simulink model "ControlThreePhaseSolarInverter"  (R2025a)
settings: Solver=VariableStepAuto  StartTime=0.0  StopTime=T  RelTol=1e-3
PreLoadFcn:
  | run('ControlThreePhaseSolarInverterParameters.m');
values from neighbouring files (symbols this model uses):
  c = 10.5e-4    (= 0.00105)    [ControlThreePhaseSolarInverterParameters.m]
  l = 1e-3    (= 0.001)    [ControlThreePhaseSolarInverterParameters.m]
  Ts = 50e-6    (= 5e-05)    [ControlThreePhaseSolarInverterParameters.m]
undefined symbols (not defined in the file or in its folder): array, grid, mPPT, panel
libraries: nesl_utility x9, ee_lib x6, fl_lib x5, eeRenewablesControl x1
settings Model: Creator=The MathWorks, Inc.  LastModifiedBy=The MathWorks, Inc.
settings DataIOCC: ExternalInput=getinputstruct(op)  InitialState=getstatestruct(op)  ReturnWorkspaceOutputs=off  SignalLoggingName=logsout_PVControllerdemo
settings OptimizationCC: ReuseModelBlockBuffer=off
settings ModelReferenceCC: EnableRefExpFcnMdlSchedulingChecks=on
settings RTWCC: GPUComputeCapability=3.5
settings SimscapeCC: SimscapeLogType=all  SimscapeLogSimulationStatistics=on  SimscapeLogName=simlog_PVControllerdemo

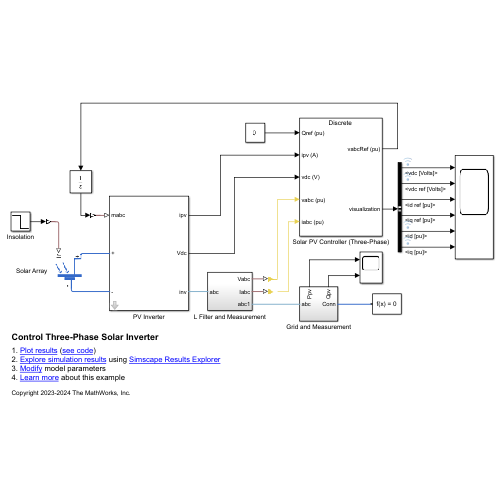
[thumbnail: Simulink's stored preview of the top-level diagram]
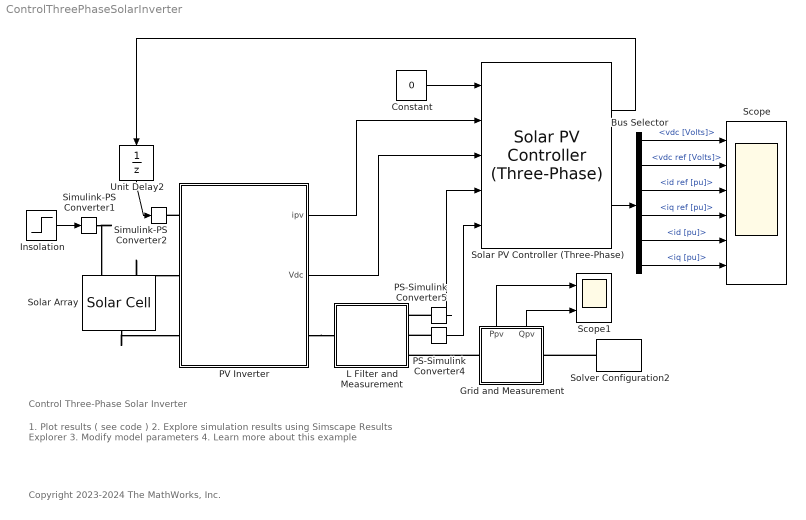
== system ControlThreePhaseSolarInverter ==
  note: 1. Plot results ( see code )
      | 2. Explore simulation results using Simscape Results Explorer
      | 3. Modify model parameters
      | 4. Learn more about this example
  note: Control Three-Phase Solar Inverter
  note: Copyright 2023-2024 The MathWorks, Inc.
  Bus Selector : BusSelector  OutputSignals=vdc [Volts],vdc ref [Volts],id ref [pu],iq ref [pu],id [pu],iq [pu]
  Constant : Constant  Value=0
  Grid and Measurement : Subsystem
      settings: PortSchema="{\"entries\":[{\"content\":{\"sides\":[{\"content\":{\"connectorIds\":[\"LConn1\"]},\"type\":\"ConnectorPlacement.EquallySpacedRectSide\",\"uuid\":\"53f3f0d9-a8a4-44c6-9152-358ba6ebb479\"},{\"content\":{\"connectorIds\":[\"RConn1\"],\"side\":\"RIGHT\"},\"type\":\"ConnectorPlacement.EquallySpacedRectSide\",\"uuid\":\"8260b293-3060-4415-851b-a3b9997b28bb\"},{\"content\":{\"connectorIds\":[\"Out1\",\"Out2\"],\"side\":\"TOP\"},\"type\":\"ConnectorPlacement.EquallySpacedRectSide\",\"uuid\":\"46e5815a-3c68-44c4-8def-43d274ad88a1\"}]},\"type\":\"ConnectorPlacement.EquallySpacedConnector\",\"uuid\":\"d7b5f747-a402-4a49-af60-c72c4c55231a\"}],\"packageUris\":[\"http://schema.mathworks.com/mf0/Connector/R2020b\"],\"version\":\"1.0\"}"
  Insolation : Step  Time=2  Before=1000  After=800  SampleTime=Ts
  L Filter and Measurement : Subsystem
  PS-Simulink Converter4 : nesl_utility/PS-Simulink Converter  PhysicalDomain=network_engine_domain  SubClassName=ps_output  LeftPortType=input  RightPortType=output  PseudoPeriodic=off  Frequencies=[]  VectorFormat=inherit  Unit=inherit  AffineConversion=off
  PS-Simulink Converter5 : nesl_utility/PS-Simulink Converter  PhysicalDomain=network_engine_domain  SubClassName=ps_output  LeftPortType=input  RightPortType=output  PseudoPeriodic=off  Frequencies=[]  VectorFormat=inherit  Unit=inherit  AffineConversion=off
  PV Inverter : Subsystem  mask{c=c, c_unit=F, g=0, g_unit=1/Ohm, vc_priority=None, vc_specify=on, vc=mPPT.initialVoltage, vc_unit=V, Pfixed=1, Pfixed_unit=W}
      mask prompts: c "Capacitance"; g "Parallel conductance"; vc_priority "Initial voltage priority"; vc_specify "Initial voltage"; vc "Initial vc"; Pfixed "Fixed power loss"
      mask TypeOptions c: Capacitor/c
      mask TypeOptions c_unit: Capacitor/c_unit
      mask TypeOptions g: Capacitor/g
      mask TypeOptions g_unit: Capacitor/g_unit
      mask TypeOptions vc_priority: Capacitor/vc_priority
      mask TypeOptions vc_specify: Capacitor/vc_specify
      mask TypeOptions vc: Capacitor/vc
      mask TypeOptions vc_unit: Capacitor/vc_unit
      mask TypeOptions Pfixed:
      | Average-Value
      | Voltage Source
      | Converter
      | (Three-Phase)/Pfixed
      mask TypeOptions Pfixed_unit:
      | Average-Value
      | Voltage Source
      | Converter
      | (Three-Phase)/Pfixed_unit
      mask DialogControl Container4 Prompt: DC Link Capacitance
      mask DialogControl Container5 Prompt: Average Inverter
  Scope : Scope  NumInputPorts=6
      settings: ActiveDisplayYMinimum=759.67451  ActiveDisplayYMaximum=881.42949
  Scope1 : Scope  NumInputPorts=2
      settings: ActiveDisplayYMinimum=-10224.92366  ActiveDisplayYMaximum=92024.31296
  Simulink-PS Converter1 : nesl_utility/Simulink-PS Converter  PhysicalDomain=network_engine_domain  SubClassName=ps_input  LeftPortType=input  RightPortType=output  PseudoPeriodic=off  Frequencies=[]  NoiseDistribution=none  NoiseParameters=[]  Unit=1  AffineConversion=off  FilteringAndDerivatives=provide  SimscapeFilterOrder=1  InputFilterTimeConstant=0.001  UdotUserProvided=0
  Simulink-PS Converter2 : nesl_utility/Simulink-PS Converter  PhysicalDomain=network_engine_domain  SubClassName=ps_input  LeftPortType=input  RightPortType=output  PseudoPeriodic=off  Frequencies=[]  NoiseDistribution=none  NoiseParameters=[]  Unit=1  AffineConversion=off  FilteringAndDerivatives=provide  SimscapeFilterOrder=1  InputFilterTimeConstant=0.001  UdotUserProvided=0
  Solar Array : ee_lib/Sources/Solar Cell  prm=3  Isc=3.8 A  Voc=0.586 V  Is=solarcell.diodeSaturationCurrent A  Is2=0 A  Iph=solarcell.solarGeneratedCurrent_AM A  Ir0=1000 W/m^2  ec=solarcell.qualityFactori  N2=solarcell.qualityFactorj  Rs=solarcell.seriesResistance Ohm  Rp=solarcell.parallelResistance Ohm  N_series=panel.nseriesCellPanel*array.nseriespanelsPerString  N_parallel=panel.nparallelStringsPanel*array.nparallelStrings  TIPH1=solarcell.tempCofficient 1/K  EG=solarcell.Eg eV  TXIS1=solarcell.temparatureExponent_Is1  TXIS2=solarcell.temparatureExponent_Is2  TRS1=solarcell.temparatureExponent_Rs  TRP1=solarcell.temparatureExponent_Rp  Tmeas=solarcell.measurementTemperature degC  TFIXED=solarcell.deviceTemperature degC  thermal_mass=100 J/K  initial_temperature=25 degC
  Solar PV Controller (Three-Phase) : eeRenewablesControl/Solar PV Controller (Three-Phase)  L=l  frequency=grid.frequency  iMax=imax  zBase=zbase  mVAbase=mVAbase  VdcBase=vdcbase  sampleTime=-1  Choice=Incremental conductance (INC)  Vdc=mPPT.initialVoltage  delV=mPPT.stepSize  tSettling=mPPT.settlingTime  Kppll=kppll  Kipll=kipll  initialPhase=0  Kpv=kpv  Kiv=kiv  Kdv=0  Kpicd=kpic  Kiicd=kiic  Kdicd=0  Kpicq=kpic  Kiicq=kiic  Kdicq=0
      settings: LibrarySourceBlock=ee_sl_lib/Renewables Control/Solar PV Controller (Three-Phase)
  Solver Configuration2 : nesl_utility/Solver Configuration  PhysicalDomain=network_engine_domain  SubClassName=solver  LeftPortType=input  RightPortType=generic  Tones=[]  Harmonics=[]  SimulateNoise=off  Profile=off  UseLocalSampling=off  EnableSwitchedLinearOptims=on  FrequencyDomain=off  UseCCode=off  RelTol=0.001  AbsTol=1e-06  MinStep=1e-09  ToWorkspace=off  RevertToSquareIcSolve=off  NumHomotopyIterations=100  PhasorMode=off  PhasorModeNumHarmonics=1  ConsistencySolver=NEWTON_FTOL  IndexReductionMethod=DerivativeReplacement  DoDC=off  ResidualTolerance=1e-09  ConsistencyTolSource=GLOBAL  ConsistencyAbsTol=0.001  ConsistencyRelTol=0.001  ConsistencyTolFactor=0.001  UseLocalSolver=on  LocalSolverChoice=NE_BACKWARD_EULER_ADVANCER  ResolveIndetEquations=on  FunctionEvalNumThread=1  LocalSolverSampleTime=Ts  DoFixedCost=on  MaxNonlinIter=3  MaxModeIter=2  ComputeImpulses=off  ImpulseIterations=2  LinearAlgebra=auto  LinearAlgebraNumThread=0  EquationFormulation=NE_TIME_EF  DelaysMemoryBudget=1024  AutomaticFiltering=on  FilteringTimeConstant=0.001  PartitionStorageMethod=EXHAUSTIVE  PartitionMemoryBudget=1024  PartitionMethod=ROBUST  MultibodyUseLocalSolver=off  MultibodyLocalSolverChoice=ODE1  MultibodyLocalSolverSampleTime=0.001
  Unit Delay2 : UnitDelay  SampleTime=Ts  HasFrameUpgradeWarning=on
  wires:
  Insolation/1 -> Simulink-PS Converter1/1
  Unit Delay2/1 -> Simulink-PS Converter2/1
  Constant/1 -> Solar PV Controller (Three-Phase)/1
  PV Inverter/1(ipv) -> Solar PV Controller (Three-Phase)/2
  PV Inverter/2(Vdc) -> Solar PV Controller (Three-Phase)/3
  PS-Simulink Converter5/1 -> Solar PV Controller (Three-Phase)/4
  PS-Simulink Converter4/1 -> Solar PV Controller (Three-Phase)/5
  Solar PV Controller (Three-Phase)/1 -> Unit Delay2/1
  Bus Selector/3 -> Scope/3  "<id ref [pu]>"
  Bus Selector/4 -> Scope/4  "<iq ref [pu]>"
  Bus Selector/6 -> Scope/6  "<iq [pu]>"
  Bus Selector/2 -> Scope/2  "<vdc ref [Volts]>"
  Bus Selector/5 -> Scope/5  "<id [pu]>"
  Solar PV Controller (Three-Phase)/2 -> Bus Selector/1
  Bus Selector/1 -> Scope/1  "<vdc [Volts]>"
  Grid and Measurement/1(Ppv) -> Scope1/1
  Grid and Measurement/2(Qpv) -> Scope1/2
  connections:
  PV Inverter/LConn1 -- Simulink-PS Converter2/RConn1
  Simulink-PS Converter1/RConn1 -- Solar Array/LConn1
  Solar Array/LConn2 -- PV Inverter/LConn2
  Solar Array/RConn1 -- PV Inverter/LConn3
  PS-Simulink Converter5/LConn1 -- L Filter and Measurement/RConn1
  PS-Simulink Converter4/LConn1 -- L Filter and Measurement/RConn2
  PV Inverter/RConn1 -- L Filter and Measurement/LConn1
  Solver Configuration2/RConn1 -- Grid and Measurement/RConn1
  Grid and Measurement/LConn1 -- L Filter and Measurement/RConn3

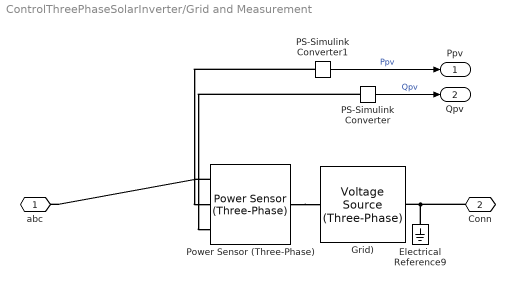
== system ControlThreePhaseSolarInverter/Grid and Measurement ==
  Electrical Reference9 : fl_lib/Electrical/Electrical Elements/Electrical Reference
  Grid) : ee_lib/Sources/Voltage Source (Three-Phase)  vline_rms=grid.voltage V  shift=0 deg  freq=grid.frequency Hz  impedance_option=0  SShortCircuit=1e6 A*V  XR=15  R=grid.Rs Ohm  L=grid.Ls H  harmonic_option=0  harmonic_orders=[5, 7, 11, 13]  harmonic_ratios=[.1, .1, .1, .1]  G_parasitic=0 1/Ohm  I_specify=off  I_priority=None  I=[0, 0, 0] A  I_nominal_specify=off  I_nominal_value=1  I_nominal_unit=A
  PS-Simulink Converter : nesl_utility/PS-Simulink Converter  PhysicalDomain=network_engine_domain  SubClassName=ps_output  LeftPortType=input  RightPortType=output  PseudoPeriodic=off  Frequencies=[]  VectorFormat=inherit  Unit=inherit  AffineConversion=off
  PS-Simulink Converter1 : nesl_utility/PS-Simulink Converter  PhysicalDomain=network_engine_domain  SubClassName=ps_output  LeftPortType=input  RightPortType=output  PseudoPeriodic=off  Frequencies=[]  VectorFormat=inherit  Unit=inherit  AffineConversion=off
  Power Sensor (Three-Phase) : ee_lib/Sensors & Transducers/Power Sensor (Three-Phase)  load_type=ee.enum.passive.type_balanced.balanced  f0=60 Hz  config=ee.enum.with_neutral.no  rho=1
      settings: InternalSimscapePortConfiguration="{\"Bottom\":[],\"Left\":[{\"id\":\"N1\",\"label\":\"~1\",\"type\":\"foundation.electrical.three_phase\"}],\"Right\":[{\"id\":\"N2\",\"label\":\"~2\",\"type\":\"foundation.electrical.three_phase\"}],\"Top\":[{\"id\":\"Pm\",\"label\":\"P\",\"type\":\"output\"},{\"id\":\"Qm\",\"label\":\"Q\",\"type\":\"output\"}]}"
  abc : PMIOPort  Side=Left
  Conn : PMIOPort  Port=2  Side=Right
  Ppv : Outport
  Qpv : Outport  Port=2
  wires:
  PS-Simulink Converter1/1 -> Ppv/1  "Ppv"
  PS-Simulink Converter/1 -> Qpv/1  "Qpv"
  connections:
  PS-Simulink Converter/LConn1 -- Power Sensor (Three-Phase)/LConn3
  PS-Simulink Converter1/LConn1 -- Power Sensor (Three-Phase)/LConn2
  Electrical Reference9/LConn1 -- Conn/RConn1 -- Grid)/LConn1
  Power Sensor (Three-Phase)/LConn1 -- abc/RConn1
  Power Sensor (Three-Phase)/RConn1 -- Grid)/RConn1

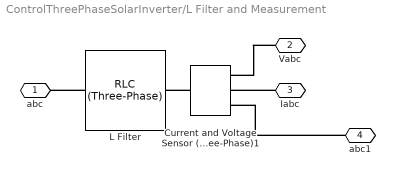
== system ControlThreePhaseSolarInverter/L Filter and Measurement ==
  Current and Voltage Sensor (Three-Phase)1 : ee_lib/Sensors & Transducers/Current and Voltage Sensor (Three-Phase)  vMeasurementType=ee.enum.vmeasurement.lg  outputUnit=ee.enum.unit.pu  SRated=mVAbase A*V  VRated=kVbase V  I_specify=off  I_priority=None  I=[0, 0, 0] A  I_nominal_specify=off  I_nominal_value=1  I_nominal_unit=A  V_specify=off  V_priority=None  V=[0, 0, 0] V  V_nominal_specify=off  V_nominal_value=1  V_nominal_unit=V
      settings: InternalSimscapePortConfiguration="{\"Bottom\":[],\"Left\":[{\"id\":\"N1\",\"label\":\"~1\",\"type\":\"foundation.electrical.three_phase\"}],\"Right\":[{\"id\":\"V_output\",\"label\":\"V\",\"type\":\"output\"},{\"id\":\"I_output\",\"label\":\"I\",\"type\":\"output\"},{\"id\":\"N2\",\"label\":\"~2\",\"type\":\"foundation.electrical.three_phase\"}],\"Top\":[]}"
  L Filter : ee_lib/Passive/RLC Assemblies/RLC (Three-Phase)  port_option=ee.enum.threePhasePort.composite  component_structure=ee.enum.rlc.structure.L  R=2e-3 Ohm  L=l H  C=1e-6 F  R_parasitic=0 Ohm  G_parasitic=0 1/Ohm  IL_specify=off  IL_priority=High  IL=[0, 0, 0] A  IL_nominal_specify=off  IL_nominal_value=1  IL_nominal_unit=A  VC_specify=off  VC_priority=High  VC=[0, 0, 0] V  VC_nominal_specify=off  VC_nominal_value=1  VC_nominal_unit=V
      settings: InternalSimscapePortConfiguration="{\"Bottom\":[],\"Left\":[{\"id\":\"N1\",\"label\":\"~1\",\"type\":\"foundation.electrical.three_phase\"}],\"Right\":[{\"id\":\"N2\",\"label\":\"~2\",\"type\":\"foundation.electrical.three_phase\"}],\"Top\":[]}"
  abc : PMIOPort  Side=Left
  Vabc : PMIOPort  Port=2  Side=Right
  Iabc : PMIOPort  Port=3  Side=Right
  abc1 : PMIOPort  Port=4  Side=Right
  connections:
  Current and Voltage Sensor (Three-Phase)1/LConn1 -- L Filter/LConn1
  Vabc/RConn1 -- Current and Voltage Sensor (Three-Phase)1/RConn1
  Iabc/RConn1 -- Current and Voltage Sensor (Three-Phase)1/RConn2
  L Filter/RConn1 -- abc/RConn1
  abc1/RConn1 -- Current and Voltage Sensor (Three-Phase)1/RConn3

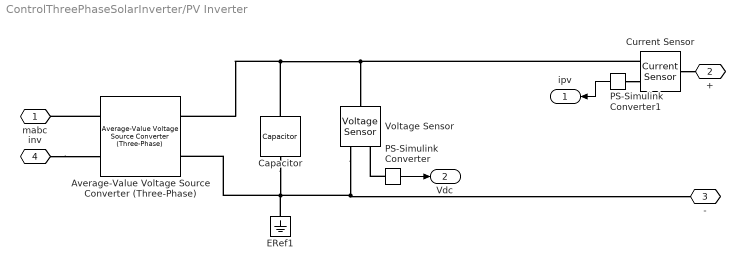
== system ControlThreePhaseSolarInverter/PV Inverter ==
  Average-Value Voltage Source Converter (Three-Phase) : ee_lib/Semiconductors & Converters/Converters/Average-Value Voltage Source Converter (Three-Phase)  port_option=ee.enum.threePhasePort.composite  frequency_option=ee.enum.converters.frequency.constant  input_option=ee.enum.converters.inputOption.ModWave  FRated=60 Hz  losses_parameterization=ee.enum.converters.losses.fixed  Pfixed=Pfixed W  ks=0.01  kc1=1.7 V  kc2=0.01 Ohm  Ploss_vect=[100, 800, 1870, 3250, 4900] W  Irms_vect=[10, 100, 200, 300, 400] A  Vdc_nom=300 V  thermal_mass=30000 J/K  temperature_specify=off  temperature_priority=High  temperature=298.15 K  temperature_nominal_specify=off  temperature_nominal_value=1  temperature_nominal_unit=K
      settings: InternalSimscapePortConfiguration="{\"Bottom\":[],\"Left\":[{\"id\":\"ModWave\",\"label\":\"ModWave\",\"type\":\"input\"},{\"id\":\"N\",\"label\":\"~\",\"type\":\"foundation.electrical.three_phase\"}],\"Right\":[{\"id\":\"p\",\"label\":\"+\",\"type\":\"foundation.electrical.electrical\"},{\"id\":\"n\",\"label\":\"-\",\"type\":\"foundation.electrical.electrical\"}],\"Top\":[]}"
  Capacitor : fl_lib/Electrical/Electrical Elements/Capacitor  c=c F  r=1e-6 Ohm  g=g 1/Ohm  i_specify=off  i_priority=None  i=0 A  i_nominal_specify=off  i_nominal_value=1  i_nominal_unit=A  v_specify=off  v_priority=None  v=6560*.5 V  v_nominal_specify=off  v_nominal_value=1  v_nominal_unit=V  vc_specify=on  vc_priority=None  vc=vc V  vc_nominal_specify=off  vc_nominal_value=1  vc_nominal_unit=V
  Current Sensor : fl_lib/Electrical/Electrical Sensors/Current Sensor
  ERef1 : fl_lib/Electrical/Electrical Elements/Electrical Reference
  PS-Simulink Converter : nesl_utility/PS-Simulink Converter  PhysicalDomain=network_engine_domain  SubClassName=ps_output  LeftPortType=input  RightPortType=output  PseudoPeriodic=off  Frequencies=[]  VectorFormat=inherit  Unit=inherit  AffineConversion=off
  PS-Simulink Converter1 : nesl_utility/PS-Simulink Converter  PhysicalDomain=network_engine_domain  SubClassName=ps_output  LeftPortType=input  RightPortType=output  PseudoPeriodic=off  Frequencies=[]  VectorFormat=inherit  Unit=inherit  AffineConversion=off
  Voltage Sensor : fl_lib/Electrical/Electrical Sensors/Voltage Sensor
  mabc : PMIOPort  Side=Left
  + : PMIOPort  Port=2  Side=Left
  - : PMIOPort  Port=3  Side=Left
  inv : PMIOPort  Port=4  Side=Right
  ipv : Outport
  Vdc : Outport  Port=2
  wires:
  PS-Simulink Converter/1 -> Vdc/1
  PS-Simulink Converter1/1 -> ipv/1
  connections:
  Voltage Sensor/RConn2 -- -/RConn1 -- ERef1/LConn1 -- Capacitor/RConn1 -- Average-Value Voltage Source Converter (Three-Phase)/RConn2
  PS-Simulink Converter/LConn1 -- Voltage Sensor/RConn1
  PS-Simulink Converter1/LConn1 -- Current Sensor/RConn1
  inv/RConn1 -- Average-Value Voltage Source Converter (Three-Phase)/LConn2
  Capacitor/LConn1 -- Current Sensor/RConn2 -- Voltage Sensor/LConn1 -- Average-Value Voltage Source Converter (Three-Phase)/RConn1
  Current Sensor/LConn1 -- +/RConn1
  Average-Value Voltage Source Converter (Three-Phase)/LConn1 -- mabc/RConn1
